simulink model "r22_switched"  (R2025b)
settings: Solver=FixedStepDiscrete  StartTime=0.0  StopTime=Tstop  FixedStep=Ts  RelTol=1e-3
values from neighbouring files (symbols this model uses):
  C = params(c)    [run_r22.m]
  Tsw = C.Tsw    [ctrl_r22.m]
undefined symbols (not defined in the file or in its folder): Ts
libraries: fl_lib x7, nesl_utility x7, ee_lib x6
settings Model: Creator=Asus ROG Strix G16  LastModifiedBy=Asus ROG Strix G16
settings DataIOCC: SaveOutput=off  SignalLogging=off  SaveTime=off

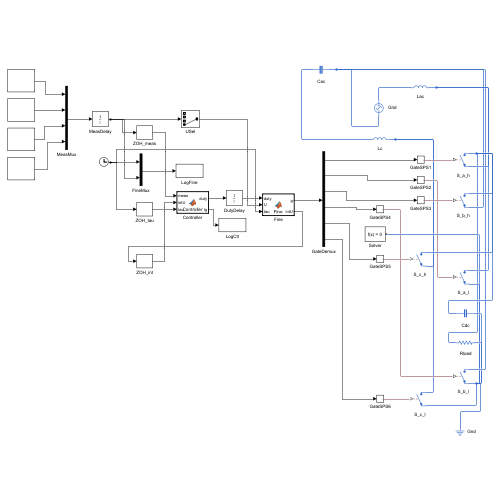
[thumbnail: Simulink's stored preview of the top-level diagram]
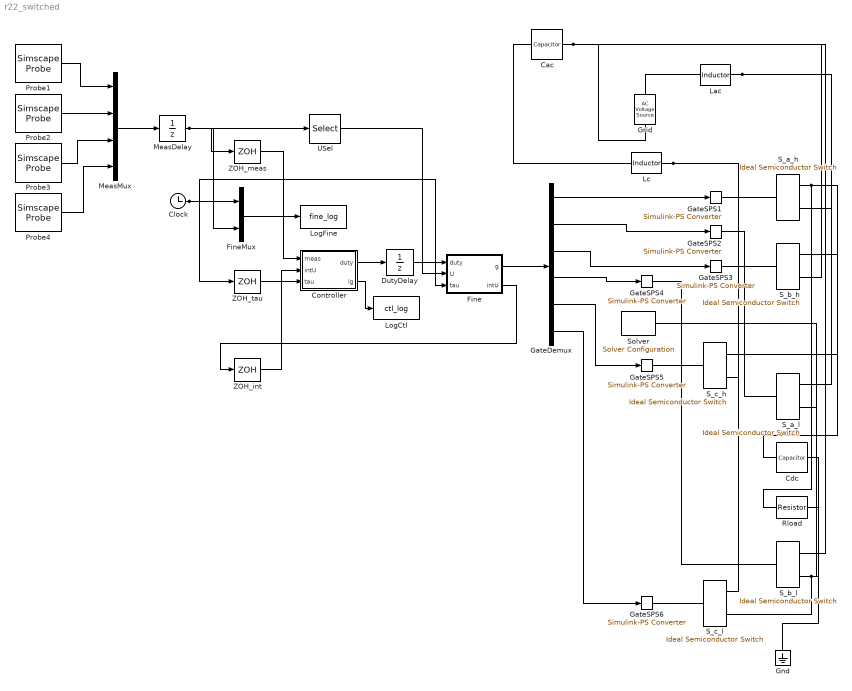
== system r22_switched ==
  Cac : fl_lib/Electrical/Electrical Elements/Capacitor  c=C.C_ac F  r=0 Ohm  g=0 1/Ohm  i_specify=off  i_priority=None  i=0 A  i_nominal_specify=off  i_nominal_value=1  i_nominal_unit=A  v_specify=off  v_priority=None  v=0 V  v_nominal_specify=off  v_nominal_value=1  v_nominal_unit=V  vc_specify=on  vc_priority=High  vc=C.uc0 V  vc_nominal_specify=off  vc_nominal_value=1  vc_nominal_unit=V
  Cdc : fl_lib/Electrical/Electrical Elements/Capacitor  c=C.C_dc F  r=0 Ohm  g=0 1/Ohm  i_specify=off  i_priority=None  i=0 A  i_nominal_specify=off  i_nominal_value=1  i_nominal_unit=A  v_specify=off  v_priority=None  v=0 V  v_nominal_specify=off  v_nominal_value=1  v_nominal_unit=V  vc_specify=on  vc_priority=High  vc=C.U0 V  vc_nominal_specify=off  vc_nominal_value=1  vc_nominal_unit=V
  Clock : Clock
  Controller : MATLAB Function  TreatAsAtomicUnit=on
  DutyDelay : UnitDelay  InitialCondition=C.duty0  SampleTime=Tsw  HasFrameUpgradeWarning=on
  Fine : MATLAB Function  TreatAsAtomicUnit=on
  FineMux : Mux  Inputs=2
  GateDemux : Demux  Outputs=6
  GateSPS{1..6} (6 alike) : nesl_utility/Simulink-PS Converter  PhysicalDomain=network_engine_domain  SubClassName=ps_input  LeftPortType=input  RightPortType=output  PseudoPeriodic=off  Frequencies=[]  NoiseDistribution=none  NoiseParameters=[]  Unit=1  AffineConversion=off  FilteringAndDerivatives=provide  SimscapeFilterOrder=1  InputFilterTimeConstant=0.001  UdotUserProvided=0
  Gnd : fl_lib/Electrical/Electrical Elements/Electrical Reference
  Grid : fl_lib/Electrical/Electrical Sources/AC Voltage Source  amp=C.U_ac V  shift=0 deg  frequency=C.f Hz
  Lac : fl_lib/Electrical/Electrical Elements/Inductor  l=C.L_ac H  r=C.R_ac Ohm  g=1e-9 1/Ohm  i_specify=off  i_priority=None  i=0 A  i_nominal_specify=off  i_nominal_value=1  i_nominal_unit=A  v_specify=off  v_priority=None  v=0 V  v_nominal_specify=off  v_nominal_value=1  v_nominal_unit=V  i_L_specify=on  i_L_priority=High  i_L=C.ia0 A  i_L_nominal_specify=off  i_L_nominal_value=1  i_L_nominal_unit=A
  Lc : fl_lib/Electrical/Electrical Elements/Inductor  l=C.L_c H  r=C.R_c Ohm  g=1e-9 1/Ohm  i_specify=off  i_priority=None  i=0 A  i_nominal_specify=off  i_nominal_value=1  i_nominal_unit=A  v_specify=off  v_priority=None  v=0 V  v_nominal_specify=off  v_nominal_value=1  v_nominal_unit=V  i_L_specify=on  i_L_priority=High  i_L=C.ic0 A  i_L_nominal_specify=off  i_L_nominal_value=1  i_L_nominal_unit=A
  LogCtl : ToWorkspace  VariableName=ctl_log  SampleTime=-1
  LogFine : ToWorkspace  VariableName=fine_log  SampleTime=-1
      settings: Decimation=fine_dec
  MeasDelay : UnitDelay  InitialCondition=C.meas0  SampleTime=Ts  HasFrameUpgradeWarning=on
  MeasMux : Mux
  Probe1 : SimscapeProbe  BoundBlock=5  Variables="{\"i_L\":{\"Probing\":\"ON\"}}"
  Probe2 : SimscapeProbe  BoundBlock=6  Variables="{\"i_L\":{\"Probing\":\"ON\"}}"
  Probe3 : SimscapeProbe  BoundBlock=7  Variables="{\"vc\":{\"Probing\":\"ON\"}}"
  Probe4 : SimscapeProbe  BoundBlock=3  Variables="{\"vc\":{\"Probing\":\"ON\"}}"
  Rload : fl_lib/Electrical/Electrical Elements/Resistor  R=C.R_load Ohm  i_specify=off  i_priority=None  i=0 A  i_nominal_specify=off  i_nominal_value=1  i_nominal_unit=A  v_specify=off  v_priority=None  v=0 V  v_nominal_specify=off  v_nominal_value=1  v_nominal_unit=V
  S_a_h : ee_lib/Semiconductors & Converters/Ideal Semiconductor Switch  port_option=ee.enum.controlport.ps  Ron=C.Ron Ohm  Goff=1e-6 1/Ohm  Vth=0.5 V  diode_param=ee.enum.converters.protectiondiode.nodynamics  diode_Vf=C.Vf V  diode_Ron=C.Ron Ohm  diode_Goff=1e-5 1/Ohm  diode_C=50e-9 F  diode_iRM=-235 A  diode_iF=300 A  diode_idot=-50 A/us  diode_trr_param=ee.enum.converters.diodetrr.trr_factor  diode_trr_factor=3  diode_trr=15 us  diode_Qrr=1500 s*uA
  S_a_l : ee_lib/Semiconductors & Converters/Ideal Semiconductor Switch  port_option=ee.enum.controlport.ps  Ron=C.Ron Ohm  Goff=1e-6 1/Ohm  Vth=0.5 V  diode_param=ee.enum.converters.protectiondiode.nodynamics  diode_Vf=C.Vf V  diode_Ron=C.Ron Ohm  diode_Goff=1e-5 1/Ohm  diode_C=50e-9 F  diode_iRM=-235 A  diode_iF=300 A  diode_idot=-50 A/us  diode_trr_param=ee.enum.converters.diodetrr.trr_factor  diode_trr_factor=3  diode_trr=15 us  diode_Qrr=1500 s*uA
  S_b_h : ee_lib/Semiconductors & Converters/Ideal Semiconductor Switch  port_option=ee.enum.controlport.ps  Ron=C.Ron Ohm  Goff=1e-6 1/Ohm  Vth=0.5 V  diode_param=ee.enum.converters.protectiondiode.nodynamics  diode_Vf=C.Vf V  diode_Ron=C.Ron Ohm  diode_Goff=1e-5 1/Ohm  diode_C=50e-9 F  diode_iRM=-235 A  diode_iF=300 A  diode_idot=-50 A/us  diode_trr_param=ee.enum.converters.diodetrr.trr_factor  diode_trr_factor=3  diode_trr=15 us  diode_Qrr=1500 s*uA
  S_b_l : ee_lib/Semiconductors & Converters/Ideal Semiconductor Switch  port_option=ee.enum.controlport.ps  Ron=C.Ron Ohm  Goff=1e-6 1/Ohm  Vth=0.5 V  diode_param=ee.enum.converters.protectiondiode.nodynamics  diode_Vf=C.Vf V  diode_Ron=C.Ron Ohm  diode_Goff=1e-5 1/Ohm  diode_C=50e-9 F  diode_iRM=-235 A  diode_iF=300 A  diode_idot=-50 A/us  diode_trr_param=ee.enum.converters.diodetrr.trr_factor  diode_trr_factor=3  diode_trr=15 us  diode_Qrr=1500 s*uA
  S_c_h : ee_lib/Semiconductors & Converters/Ideal Semiconductor Switch  port_option=ee.enum.controlport.ps  Ron=C.Ron Ohm  Goff=1e-6 1/Ohm  Vth=0.5 V  diode_param=ee.enum.converters.protectiondiode.nodynamics  diode_Vf=C.Vf V  diode_Ron=C.Ron Ohm  diode_Goff=1e-5 1/Ohm  diode_C=50e-9 F  diode_iRM=-235 A  diode_iF=300 A  diode_idot=-50 A/us  diode_trr_param=ee.enum.converters.diodetrr.trr_factor  diode_trr_factor=3  diode_trr=15 us  diode_Qrr=1500 s*uA
  S_c_l : ee_lib/Semiconductors & Converters/Ideal Semiconductor Switch  port_option=ee.enum.controlport.ps  Ron=C.Ron Ohm  Goff=1e-6 1/Ohm  Vth=0.5 V  diode_param=ee.enum.converters.protectiondiode.nodynamics  diode_Vf=C.Vf V  diode_Ron=C.Ron Ohm  diode_Goff=1e-5 1/Ohm  diode_C=50e-9 F  diode_iRM=-235 A  diode_iF=300 A  diode_idot=-50 A/us  diode_trr_param=ee.enum.converters.diodetrr.trr_factor  diode_trr_factor=3  diode_trr=15 us  diode_Qrr=1500 s*uA
  Solver : nesl_utility/Solver Configuration  PhysicalDomain=network_engine_domain  SubClassName=solver  LeftPortType=input  RightPortType=generic  Tones=[]  Harmonics=[]  SimulateNoise=off  Profile=off  UseLocalSampling=off  EnableSwitchedLinearOptims=on  FrequencyDomain=off  UseCCode=off  RelTol=0.001  AbsTol=0.001  MinStep=1e-09  ToWorkspace=off  RevertToSquareIcSolve=off  NumHomotopyIterations=100  PhasorMode=off  PhasorModeNumHarmonics=1  ConsistencySolver=NEWTON_XTOL_AFTER_FTOL  IndexReductionMethod=DerivativeReplacement  DoDC=off  ResidualTolerance=1e-09  ConsistencyTolSource=GLOBAL  ConsistencyAbsTol=0.001  ConsistencyRelTol=0.001  ConsistencyTolFactor=0.001  UseLocalSolver=on  LocalSolverChoice=NE_PARTITIONING_ADVANCER  ResolveIndetEquations=on  FunctionEvalNumThread=1  LocalSolverSampleTime=Ts  DoFixedCost=on  MaxNonlinIter=3  MaxModeIter=2  ComputeImpulses=off  ImpulseIterations=2  LinearAlgebra=auto  LinearAlgebraNumThread=0  EquationFormulation=NE_TIME_EF  DelaysMemoryBudget=1024  AutomaticFiltering=on  FilteringTimeConstant=0.001  PartitionStorageMethod=AS_NEEDED  PartitionMemoryBudget=1024  PartitionMethod=ROBUST  MultibodyUseLocalSolver=off  MultibodyLocalSolverChoice=ODE1  MultibodyLocalSolverSampleTime=0.001
  USel : Selector  InputPortWidth=4  IndexOptions=Index vector (dialog)  Indices=4  OutputSizes=1
  ZOH_int : ZeroOrderHold  SampleTime=Tsw
  ZOH_meas : ZeroOrderHold  SampleTime=Tsw
  ZOH_tau : ZeroOrderHold  SampleTime=Tsw
  wires:
  USel/1 -> Fine/2(U)
  MeasMux/1 -> MeasDelay/1
  Probe1/1 -> MeasMux/1
  Clock/1 -> Fine/3(tau), ZOH_tau/1, FineMux/1
  Probe2/1 -> MeasMux/2
  Probe3/1 -> MeasMux/3
  MeasDelay/1 -> ZOH_meas/1, FineMux/2, USel/1
  Probe4/1 -> MeasMux/4
  ZOH_meas/1 -> Controller/1(meas)
  FineMux/1 -> LogFine/1
  ZOH_tau/1 -> Controller/3(tau)
  ZOH_int/1 -> Controller/2(intU)
  Controller/1(duty) -> DutyDelay/1
  Controller/2(lg) -> LogCtl/1
  DutyDelay/1 -> Fine/1(duty)
  Fine/1(g) -> GateDemux/1
  Fine/2(intU) -> ZOH_int/1
  GateDemux/4 -> GateSPS4/1
  GateDemux/1 -> GateSPS1/1
  GateDemux/2 -> GateSPS2/1
  GateDemux/3 -> GateSPS3/1
  GateDemux/5 -> GateSPS5/1
  GateDemux/6 -> GateSPS6/1
  connections:
  GateSPS2/RConn1 -- S_a_l/LConn1
  GateSPS4/RConn1 -- S_b_l/LConn1
  Cac/LConn1 -- Lc/LConn1
  Cac/RConn1 -- Grid/RConn1 -- S_b_l/RConn1 -- S_b_h/RConn2
  GateSPS6/RConn1 -- S_c_l/LConn1
  Grid/LConn1 -- Lac/LConn1
  Lc/RConn1 -- S_c_h/RConn2 -- S_c_l/RConn1
  GateSPS5/RConn1 -- S_c_h/LConn1
  Lac/RConn1 -- S_a_h/RConn2 -- S_a_l/RConn1
  GateSPS1/RConn1 -- S_a_h/LConn1
  GateSPS3/RConn1 -- S_b_h/LConn1
  S_c_h/RConn1 -- S_b_h/RConn1 -- S_a_h/RConn1 -- Rload/LConn1 -- Cdc/LConn1
  S_c_l/RConn2 -- S_a_l/RConn2 -- Gnd/LConn1 -- Cdc/RConn1 -- Rload/RConn1 -- Solver/RConn1 -- S_b_l/RConn2

== matlab function r22_switched/Controller ==
  data: meas input; duty output; intU input; tau input; lg output; C parameter
function [duty, lg] = Controller(meas, intU, tau, C)
%#codegen
[duty, lg] = ctrl_r22(meas, intU, tau, C);

== matlab function r22_switched/Fine ==
  data: duty input; g output; U input; tau input; intU output; C parameter
function [g, intU] = Fine(duty, U, tau, C)
%#codegen
[g, intU] = fine_r22(duty, U, tau, C);
